simulink model "turbo_controller"  (R2025a)
settings: Solver=FixedStepAuto  StartTime=0.0  StopTime=inf  FixedStep=0.001  RelTol=1e-3
PostLoadFcn:
  | % 自动定位同目录CubeMX文件；不需要外部初始化脚本。
  | codertarget.data.setParameterValue('turbo_controller','STM32CubeMX.ProjectFile',fullfile(fileparts(get_param('turbo_controller','FileName')),'turbo_f407.ioc'));
InitFcn:
  | % 中文说明：按原控制器字段与类型创建三组接口总线；控制参数已内嵌。
  | tc_names=["EValve_Cycle" "EValve_Open" "Eblast_Cycle" "Eblast_Open" "Motor_Cycle" "Motor_Open" "EValve_Enable" "Eblast_Enable" "Motor_Enable" "SWO_Firework" "SWO_BleedAir" "EngineState" "Flag_ECUReset_Clear" "Flag_ECUReset_Save" "Flag_Reset_Enable" "Accelerator" "Nc_dem" "Nc"]; tc_types=["uint16" "uint16" "uint16" "uint16" "uint16" "uint16" "uint8" "uint8" "uint8" "uint8" "uint8" "uint8" "uint8" "uint8" "uint8" "single" "single" "single"];
  | for tc_k=1:numel(tc_names)
  |  tc_e(tc_k)=Simulink.BusElement; tc_e(tc_k).Name=char(tc_names(tc_k)); tc_e(tc_k).DataType=char(tc_types(tc_k));
  | end
  | EngineControl_Out=Simulink.Bus; EngineControl_Out.DataScope='Exported'; EngineControl_Out.Elements=tc_e;
  | clear tc_e tc_names tc_types tc_k
  | tc_names=["savedata1" "savedata2" "savedata3" "savedata4" "savedata5" "savedata6" "savedata7" "savedata8" "savedata9" "savedata10" "savedata11" "savedata12" "savedata13" "savedata14" "savedata15" "savedata16" "savedata17" "savedata18" "savedata19" "savedata20" "savedata21" "savedata22" "savedata23" "savedata24" "savedata25"]; tc_types=["single" "single" "single" "single" "single" "single" "single" "single" "single" "single" "single" "single" "single" "single" "single" "single" "single" "single" "single" "single" "single" "single" "single" "single" "single"];
  | for tc_k=1:numel(tc_names)
  |  tc_e(tc_k)=Simulink.BusElement; tc_e(tc_k).Name=char(tc_names(tc_k)); tc_e(tc_k).DataType=char(tc_types(tc_k));
  | end
  | SaveData_Out=Simulink.Bus; SaveData_Out.DataScope='Exported'; SaveData_Out.Elements=tc_e;
  | clear tc_e tc_names tc_types tc_k
  | tc_names=["senddata1" "senddata2" "senddata3" "senddata4" "senddata5" "senddata6" "senddata7" "senddata8" "senddata9" "senddata10" "senddata11" "senddata12" "senddata13" "senddata14" "senddata15" "senddata16" "senddata17" "senddata18" "senddata19" "senddata20" "senddata21" "senddata22" "senddata23" "senddata24" "senddata25" "senddata26" "senddata27" "senddata28" "senddata29"]; tc_types=["uint8" "uint8" "uint8" "uint8" "uint8" "uint8" "uint8" "uint8" "uint8" "uint8" "uint8" "uint8" "uint8" "uint8" "uint8" "uint8" "uint8" "uint8" "uint8" "uint8" "uint8" "uint8" "uint8" "uint8" "uint8" "uint8" "uint8" "uint8" "uint8"];
  | for tc_k=1:numel(tc_names)
  |  tc_e(tc_k)=Simulink.BusElement; tc_e(tc_k).Name=char(tc_names(tc_k)); tc_e(tc_k).DataType=char(tc_types(tc_k));
  | end
  | SendData_Out=Simulink.Bus; SendData_Out.DataScope='Exported'; SendData_Out.Elements=tc_e;
  | clear tc_e tc_names tc_types tc_k
  | 
  | % 以下为接口中文说明；只设置描述，不改变数值或数据类型。
  | EngineControl_Out.Description='执行控制输出（阀、电机、点火、状态及复位请求）';
  | tc_cn=["EValve_Cycle（主油阀周期计数（每计数2毫秒））" "EValve_Open（主油阀开通计数（每计数2毫秒））" "Eblast_Cycle（副油阀周期计数（每计数2毫秒））" "Eblast_Open（副油阀开通计数（每计数2毫秒））" "Motor_Cycle（起动电机周期计数）" "Motor_Open（起动电机开通计数）" "EValve_Enable（主油阀驱动使能）" "Eblast_Enable（副油阀驱动使能）" "Motor_Enable（起动电机使能）" "SWO_Firework（点火器使能（1开））" "SWO_BleedAir（引气阀使能（1开））" "EngineState（发动机状态）" "Flag_ECUReset_Clear（清除复位恢复状态请求）" "Flag_ECUReset_Save（保存复位恢复数据请求）" "Flag_Reset_Enable（处理器软件复位请求）" "Accelerator（油门／油泵给定控制量）" "Nc_dem（控制目标转速）" "Nc（发动机反馈转速（转每分））"];
  | tc_elements=EngineControl_Out.Elements;
  | for tc_k=1:numel(tc_cn)
  |  tc_elements(tc_k).Description=char(tc_cn(tc_k));
  | end
  | EngineControl_Out.Elements=tc_elements;
  | clear tc_cn tc_elements tc_k
  | SaveData_Out.Description='25项运行记录；字段含义按当前模型数据来源解释';
  | tc_cn=["savedata1（指令回显记录）" "savedata2（入口总温记录（℃））" "savedata3（电源电压记录）" "savedata4（排气温度记录（℃））" "savedata5（标定燃油压力记录）" "savedata6（副油阀占空比记录（％））" "savedata7（主油阀占空比记录（％））" "savedata8（温度修正转速记录）" "savedata9（开关输出及反馈位域）" "savedata10（物理转速记录）" "savedata11（油泵目标给定原始值）" "savedata12（起动电机占空比记录（％））" "savedata13（发动机状态码记录）" "savedata14（故障告警位域记录）" "savedata15（模型记录帧序号）" "savedata16（处理器温度记录（℃））" "savedata17（装订转速记录（沿用旧电源字段名））" "savedata18（导航高度记录）" "savedata19（飞行空速记录）" "savedata20（主阀旧记录位（恒零保留））" "savedata21（第21项保留记录（恒零））" "savedata22（保留记录项22）" "savedata23（保留记录项23）" "savedata24（保留记录项24）" "savedata25（保留记录项25）"];
  | tc_elements=SaveData_Out.Elements;
  | for tc_k=1:numel(tc_cn)
  |  tc_elements(tc_k).Description=char(tc_cn(tc_k));
  | end
  | SaveData_Out.Elements=tc_elements;
  | clear tc_cn tc_elements tc_k
  | SendData_Out.Description='29字段回传及外设命令接口；板端上位机帧只取第3至27字段';
  | tc_cn=["senddata1（回传发送允许标志（不直接上线路））" "senddata2（回传载荷长度25字节）" "senddata3（回传指令回显字节）" "senddata4（总温编码字节（℃＋80））" "senddata5（电源电压编码字节）" "senddata6（排温编码高字节）" "senddata7（排温编码低字节）" "senddata8（燃油压力编码高字节）" "senddata9（燃油压力编码低字节）" "senddata10（副油阀占空比字节（％））" "senddata11（主油阀占空比字节（％））" "senddata12（修正转速编码高字节）" "senddata13（修正转速编码低字节）" "senddata14（驱动及反馈状态位域）" "senddata15（物理转速编码高字节）" "senddata16（物理转速编码低字节）" "senddata17（油泵目标给定高字节（串口二使用））" "senddata18（油泵目标给定低字节（串口二使用））" "senddata19（起动电机占空比命令（串口一使用））" "senddata20（发动机状态码字节）" "senddata21（故障告警位域字节）" "senddata22（帧序号占位（板端另行填写））" "senddata23（处理器温度编码（℃＋50））" "senddata24（控制目标转速编码高字节）" "senddata25（控制目标转速编码低字节）" "senddata26（占位字节（板端改填实测泵速高字节））" "senddata27（占位字节（板端改填实测泵速低字节））" "senddata28（装订转速高字节（本板未发送））" "senddata29（装订转速低字节（本板未发送））"];
  | tc_elements=SendData_Out.Elements;
  | for tc_k=1:numel(tc_cn)
  |  tc_elements(tc_k).Description=char(tc_cn(tc_k));
  | end
  | SendData_Out.Elements=tc_elements;
  | clear tc_cn tc_elements tc_k
  | 
  | 
  | % FRAM模块化事务：接口类型和上电初始状态，随模型保存，无外部初始化文件。
  | clear FM_elements
  | FM_elements(1)=Simulink.BusElement;FM_elements(1).Name='phase';FM_elements(1).DataType='uint8';FM_elements(1).Dimensions=[1 1];FM_elements(1).Description='phase（当前事务阶段）';
  | FM_elements(2)=Simulink.BusElement;FM_elements(2).Name='a';FM_elements(2).DataType='uint8';FM_elements(2).Dimensions=[64 1];FM_elements(2).Description='a（启动时缓存的首区64字节）';
  | FM_elements(3)=Simulink.BusElement;FM_elements(3).Name='active';FM_elements(3).DataType='uint16';FM_elements(3).Dimensions=[1 1];FM_elements(3).Description='active（当前有效记录区地址）';
  | FM_elements(4)=Simulink.BusElement;FM_elements(4).Name='generation';FM_elements(4).DataType='uint32';FM_elements(4).Dimensions=[1 1];FM_elements(4).Description='generation（当前有效记录代号）';
  | FM_elements(5)=Simulink.BusElement;FM_elements(5).Name='record';FM_elements(5).DataType='uint8';FM_elements(5).Dimensions=[64 1];FM_elements(5).Description='record（本次冻结的待写记录）';
  | FM_elements(6)=Simulink.BusElement;FM_elements(6).Name='addr';FM_elements(6).DataType='uint16';FM_elements(6).Dimensions=[1 1];FM_elements(6).Description='addr（本次备用写入地址）';
  | FM_elements(7)=Simulink.BusElement;FM_elements(7).Name='lastSave';FM_elements(7).DataType='single';FM_elements(7).Dimensions=[1 1];FM_elements(7).Description='lastSave（上次开始保存的秒数）';
  | FM_elements(8)=Simulink.BusElement;FM_elements(8).Name='lastState';FM_elements(8).DataType='uint8';FM_elements(8).Dimensions=[1 1];FM_elements(8).Description='lastState（上次保存时的发动机状态）';
  | FM_elements(9)=Simulink.BusElement;FM_elements(9).Name='boot';FM_elements(9).DataType='boolean';FM_elements(9).Dimensions=[1 1];FM_elements(9).Description='boot（启动记录是否允许恢复）';
  | FM_elements(10)=Simulink.BusElement;FM_elements(10).Name='consumed';FM_elements(10).DataType='boolean';FM_elements(10).Dimensions=[1 1];FM_elements(10).Description='consumed（本次启动恢复通知是否已发送）';
  | FM_elements(11)=Simulink.BusElement;FM_elements(11).Name='payload';FM_elements(11).DataType='uint8';FM_elements(11).Dimensions=[20 1];FM_elements(11).Description='payload（当前20字节恢复内容）';
  | ... (+35 lines)
model workspace (MAT data in the model file):
  CRC16_Table_Reference = [0 4129 8258 12387 16516 20645 24774 28903 33032 37161 41290 45419 ... (256 elements, 256x1)]
  PE_Kaer = [0.15402 0.15402 0.12264 0.10076 0.09481 0.07601 0.07111 0.0569 0.05198 0.04926 0.05308 0.04325 ... (13 elements, 1x13)]
  PE_Nr = [21.2982 61.4260372 67.7475458 72.7394382 76.845934 80.6988798 83.8449282 86.6491912 88.9382406 89.178606 91.1938214 93.4068058 ... (13 elements, 1x13)]
  PE_Pump_Translate = 33.5999984741
  PE_RotaSpeed_Translate = 860
  PE_Taer = [0.4939154 0.4939154 0.40780982 0.34066978 0.31622756 0.30405716 0.34300244 0.26785022 0.37393554 0.23914836 0.44563948 0.31044662 ... (13 elements, 1x13)]
  PF_ACCFULLRANGE = 3360
  PF_Flag_ECUReset = 0
  PF_Flag_rx_suc = 1
  PF_Gear_Info = [40000; 45000; 50000; 55000; 57000; 59000; 60000; 61000; 61000; 61000; 61000; 61000]
  PF_K_TiaoJie = 1
  PF_Kpu = 10
  PF_MySet_Rxdata = [0 0 0 0 0 0 0 0 0 0 0 0 ... (50 elements, 50x1)]
  PF_MyUsart1_Rxdata = [0 0 0 0 0 0 0 0 0 0 0 0 ... (50 elements, 50x1)]
  PF_MyUsart2_Rxdata = [0 0 0 0 0 0 0 0 0 0 0 0 ... (50 elements, 50x1)]
  PF_Reset_Information = [0 0 0 0 0 0 0 0 0 0 0 0 ... (20 elements, 20x1)]
  PF_Sensor_X1_T4 = [0 4095]
  PF_Sensor_X2_T4 = [0 1.66666698456]
  PF_Sensor_X3_T4 = [0 504 999 1497 2010 2529 3051 3568 4076 4571 4959]
  PF_Sensor_X_P2 = [0.5 3]
  PF_Sensor_X_Poil = [0.5 3]
  PF_Sensor_X_T1t = [-50 300]
  PF_Sensor_X_Vpower = [0 3]
  PF_Sensor_X_Vpump = [0 3]
  PF_Sensor_Y1_T4 = [0 3]
  PF_Sensor_Y2_T4 = [0 5000]
  PF_Sensor_Y3_T4 = [0 100 200 300 400 500 600 700 800 900 980]
  PF_Sensor_Y_P2 = [0 1000]
  PF_Sensor_Y_Poil = [0 1000]
  PF_Sensor_Y_T1t = [-50 300]
  PF_Sensor_Y_Vpower = [0 33]
  PF_Sensor_Y_Vpump = [0 33]
  PG_CtrlMode_CloseLoop : mpt.Parameter (value not decoded)
  PG_CtrlMode_ManualAcc : mpt.Parameter (value not decoded)
  PG_CtrlMode_Origin : mpt.Parameter (value not decoded)
  PG_CtrlMode_Start : mpt.Parameter (value not decoded)
  PG_CtrlMode_Stop : mpt.Parameter (value not decoded)
  PG_ES_Clp : mpt.Parameter (value not decoded)
  PG_ES_EngStart : mpt.Parameter (value not decoded)
  PG_ES_Manual : mpt.Parameter (value not decoded)
  PG_ES_Origin : mpt.Parameter (value not decoded)
  PG_ES_Stop : mpt.Parameter (value not decoded)
  PG_Instr_BleedAirSet : mpt.Parameter (value not decoded)
  PG_Instr_CloseLoop : mpt.Parameter (value not decoded)
  PG_Instr_ECUReSet : mpt.Parameter (value not decoded)
  PG_Instr_EValveSet : mpt.Parameter (value not decoded)
  PG_Instr_EblastSet : mpt.Parameter (value not decoded)
  PG_Instr_Erase : mpt.Parameter (value not decoded)
  PG_Instr_FireWorkSet : mpt.Parameter (value not decoded)
  PG_Instr_ManualPlus : mpt.Parameter (value not decoded)
  PG_Instr_ManualrReduce : mpt.Parameter (value not decoded)
  PG_Instr_MotorSet : mpt.Parameter (value not decoded)
  PG_Instr_OilSet : mpt.Parameter (value not decoded)
  PG_Instr_SelfCheck : mpt.Parameter (value not decoded)
  PG_Instr_Start : mpt.Parameter (value not decoded)
  PG_Instr_Stop : mpt.Parameter (value not decoded)
  PG_Instr_StopZero : Simulink.Parameter (value not decoded)
  PG_Location_Air : Simulink.Parameter (value not decoded)
  PG_Location_Gnd : Simulink.Parameter (value not decoded)
  PG_ServoCtrlMode_CloseLoop : Simulink.Parameter (value not decoded)
  PG_ServoCtrlMode_CloseLoopMax : Simulink.Parameter (value not decoded)
  PG_ServoCtrlMode_CloseLoopMin : Simulink.Parameter (value not decoded)
  PG_ServoCtrlMode_ManualAcc : Simulink.Parameter (value not decoded)
  PG_ServoCtrlMode_ManualAccMax : Simulink.Parameter (value not decoded)
  PG_ServoCtrlMode_ManualAccMin : Simulink.Parameter (value not decoded)
  PG_SpeedDot_Permit : Simulink.Parameter (value not decoded)
  PL_EngineModel_Actuator = [0 10 100]
  PL_EngineModel_EngineStar_Press_P2 = [1013 1098.4 1099.144828 1099.931034 1103.613793 1162.662069 1143.793103 1131.006897 1123.186207 1117.6 1114 1111.806897 ... (127 elements, 1x127)]
  PL_EngineModel_EngineStar_RotaSpeed = [200 2000 9584 9660 10220 10240 10260 10288 10308 10368 10380 10408 ... (127 elements, 1x127)]
  PL_EngineModel_EngineStar_Temp_Exhaust = [128 129 129.1 130 131 131.1 132 133 134 134.1 135 135.1 ... (127 elements, 1x127)]
  PL_EngineModel_EngineStar_Time = [0.05 0.1 0.15 0.2 0.25 0.3 0.35 0.4 0.45 0.5 0.55 0.6 ... (127 elements, 1x127)]
  PL_EngineModel_IdleAbove_Nr = [0 21.2982 61.4260372 67.7475458 72.7394382 76.845934 80.6988798 83.8449282 86.6491912 88.9382406 89.178606 91.1938214 ... (14 elements, 1x14)]
  PL_EngineModel_IdleAbove_P2r = [0.986923266716 1.57907722675 1.81593881076 1.99358499877 2.23044658278 2.43770046879 2.65482358747 2.84233900814 3.03972366149 3.18776215149 3.25684678016 3.3950160375 ... (14 elements, 1x14)]
  PL_EngineModel_IdleAbove_Tempr = [0.0536001429337 1.07200285867 1.63301768805 1.63659103091 1.66875111667 1.72592460247 1.77595140254 1.86171163123 1.95461854565 2.03323208862 2.03323208862 2.13685903162 ... (14 elements, 1x14)]
  PL_EngineModel_IdleAbove_Ter = [0.42434128 0.42434128 0.42434128 0.30669408 0.23570008 0.22150128 0.1997974 0.23803274 0.16115638 0.24279948 0.13600422 0.31308354 ... (14 elements, 1x14)]
  PL_EngineModel_IdleAbove_Wfr = [0 10.142 23.8337 27.8905 31.9473 36.0041 40.0609 44.1177 48.1745 52.2313 52.7384 56.7952 ... (14 elements, 1x14)]
  PL_EngineModel_Press_P2 = [400 400 400 400 400 400 400 400 400 400]
  PL_EngineModel_Rotaspeed = [0 20000 96400]
  PL_EngineModel_Temp_Exhaust = [500 500 500 500 500 500 500 500 500 500]
  PL_Kaer = [0.1 0.1 0.1 0.1 0.1 0.1]
  PL_Nr = [50 60 70 80 90 100]
  PL_Taer = [0.1 0.1 0.1 0.1 0.1 0.1]
  Sig : Simulink.Signal (value not decoded)
  Ts_ms : Simulink.Parameter (value not decoded)
  false : Simulink.Parameter (value not decoded)
  true : Simulink.Parameter (value not decoded)
symbols that are objects in the model workspace (value not decoded): PG_CtrlMode_CloseLoop, PG_CtrlMode_ManualAcc, PG_CtrlMode_Origin, PG_CtrlMode_Start, PG_CtrlMode_Stop, PG_ES_Clp, PG_ES_EngStart, PG_ES_Manual, PG_ES_Origin, PG_ES_Stop, PG_Instr_BleedAirSet, PG_Instr_CloseLoop, PG_Instr_EblastSet, PG_Instr_ECUReSet, PG_Instr_Erase, PG_Instr_EValveSet, PG_Instr_FireWorkSet, PG_Instr_ManualPlus, PG_Instr_ManualrReduce, PG_Instr_MotorSet, PG_Instr_OilSet, PG_Instr_SelfCheck, PG_Instr_Start, PG_Instr_Stop, PG_Instr_StopZero, PG_ServoCtrlMode_CloseLoop, PG_ServoCtrlMode_CloseLoopMax, PG_ServoCtrlMode_CloseLoopMin, PG_ServoCtrlMode_ManualAcc, PG_ServoCtrlMode_ManualAccMax, PG_ServoCtrlMode_ManualAccMin, Ts_ms
libraries: simulink x97, stm32blockslib x10, stm32f4xxblockslib x8
(part 3 of 26)

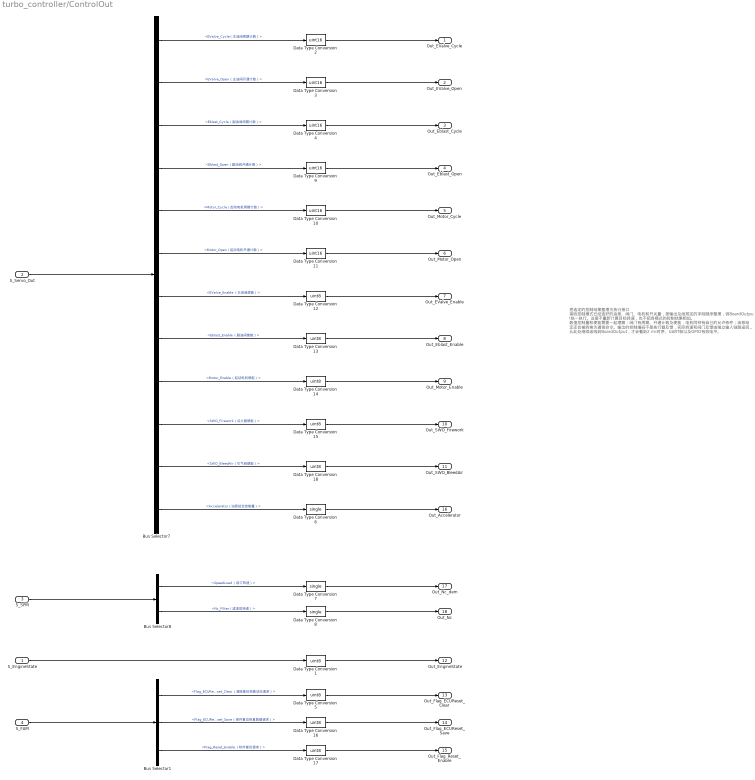
== system turbo_controller/ControlOut ==
  note: 把选定的控制结果整理为执行接口
      |
      | 接收控制模式已经选好的油泵、阀门、电机和开关量，按输出总线规定的字段顺序整理，供BoardOutpu
      | t统一执行。这里不重新计算目标转速，也不把各模式的控制结果相加。
      |
      | 数值控制量和使能需要一起理解：阀门有周期、开通计数及使能，电机同样有自己的允许条件；油泵给
      | 定还会被转换为通信命令。输出的控制编码不是执行器反馈，实际转速和阀门反馈由独立输入链路返回
      | 。
      |
      | 从此处继续追线到BoardOutput，才会看到2 ms时序、UART帧以及GPIO有效电平。
  S_EngineState : Inport
      settings: AttributesFormatString=S_EngineState（发动机状态）
  S_Servo_Out : Inport  Port=2
      settings: AttributesFormatString=S_Servo_Out（伺服输出）
  S_SPM : Inport  Port=3
      settings: AttributesFormatString=S_SPM（通信及传感器信息总线）
  S_FAM : Inport  Port=4
      settings: AttributesFormatString=S_FAM（故障标志总线）
  Bus Selector1 : BusSelector  OutputSignals=Flag_ECUReset_Clear（清除复位恢复状态请求）,Flag_ECUReset_Save（保存复位恢复数据请求）,Flag_Reset_Enable（软件复位请求）
      settings: AttributesFormatString=Bus Selector1（总线选择器1）
  Bus Selector7 : BusSelector  OutputSignals=EValve_Cycle（主油阀周期计数）,EValve_Open（主油阀开通计数）,Eblast_Cycle（副油阀周期计数）,Eblast_Open（副油阀开通计数）,Motor_Cycle（起动电机周期计数）,Motor_Open（起动电机开通计数）,EValve_Enable（主油阀使能）,Eblast_Enable（副油阀使能）,Motor_Enable（起动电机使能）,SWO_Firework（点火器使能）,SWO_BleedAir（引气阀使能）,Accelerator（油泵给定控制量）
      settings: AttributesFormatString=Bus Selector7（总线选择器7）
  Bus Selector8 : BusSelector  OutputSignals=COMM（通信信息总线）.SpeedLoad（装订转速）,Sensor（传感器信息总线）.Nc_Filter（滤波后转速）
      settings: AttributesFormatString=Bus Selector8（总线选择器8）
  Data Type Conversion{1,5,12..18} (9 alike) : DataTypeConversion  OutDataTypeStr=uint8  SaturateOnIntegerOverflow=off  RndMeth=Floor
      Data Type Conversion1 settings: AttributesFormatString=Data Type Conversion1（数据类型转换1）
      Data Type Conversion12 settings: AttributesFormatString=Data Type Conversion12（数据类型转换12）
      Data Type Conversion13 settings: AttributesFormatString=Data Type Conversion13（数据类型转换13）
      Data Type Conversion14 settings: AttributesFormatString=Data Type Conversion14（数据类型转换14）
      Data Type Conversion15 settings: AttributesFormatString=Data Type Conversion15（数据类型转换15）
      Data Type Conversion16 settings: AttributesFormatString=Data Type Conversion16（数据类型转换16）
      Data Type Conversion17 settings: AttributesFormatString=Data Type Conversion17（数据类型转换17）
      Data Type Conversion18 settings: AttributesFormatString=Data Type Conversion18（数据类型转换18）
      Data Type Conversion5 settings: AttributesFormatString=Data Type Conversion5（数据类型转换5）
  Data Type Conversion{2..4,9..11} (6 alike) : DataTypeConversion  OutDataTypeStr=uint16  SaturateOnIntegerOverflow=off  RndMeth=Floor
      Data Type Conversion10 settings: AttributesFormatString=Data Type Conversion10（数据类型转换10）
      Data Type Conversion11 settings: AttributesFormatString=Data Type Conversion11（数据类型转换11）
      Data Type Conversion2 settings: AttributesFormatString=Data Type Conversion2（数据类型转换2）
      Data Type Conversion3 settings: AttributesFormatString=Data Type Conversion3（数据类型转换3）
      Data Type Conversion4 settings: AttributesFormatString=Data Type Conversion4（数据类型转换4）
      Data Type Conversion9 settings: AttributesFormatString=Data Type Conversion9（数据类型转换9）
  Data Type Conversion6 : DataTypeConversion  OutDataTypeStr=single  SaturateOnIntegerOverflow=off  RndMeth=Floor
      settings: AttributesFormatString=Data Type Conversion6（数据类型转换6）
  Data Type Conversion7 : DataTypeConversion  OutDataTypeStr=single  SaturateOnIntegerOverflow=off  RndMeth=Floor
      settings: AttributesFormatString=Data Type Conversion7（数据类型转换7）
  Data Type Conversion8 : DataTypeConversion  OutDataTypeStr=single  SaturateOnIntegerOverflow=off  RndMeth=Floor
      settings: AttributesFormatString=Data Type Conversion8（数据类型转换8）
  Out_EValve_Cycle : Outport
      settings: AttributesFormatString=Out_EValve_Cycle（主油阀周期计数（每计数2毫秒））
  Out_EValve_Open : Outport  Port=2
      settings: AttributesFormatString=Out_EValve_Open（主油阀开通计数（每计数2毫秒））
  Out_Eblast_Cycle : Outport  Port=3
      settings: AttributesFormatString=Out_Eblast_Cycle（副油阀周期计数（每计数2毫秒））
  Out_Eblast_Open : Outport  Port=4
      settings: AttributesFormatString=Out_Eblast_Open（副油阀开通计数（每计数2毫秒））
  Out_Motor_Cycle : Outport  Port=5
      settings: AttributesFormatString=Out_Motor_Cycle（起动电机周期计数）
  Out_Motor_Open : Outport  Port=6
      settings: AttributesFormatString=Out_Motor_Open（起动电机开通计数）
  Out_EValve_Enable : Outport  Port=7
      settings: AttributesFormatString=Out_EValve_Enable（主油阀驱动使能）
  Out_Eblast_Enable : Outport  Port=8
      settings: AttributesFormatString=Out_Eblast_Enable（副油阀驱动使能）
  Out_Motor_Enable : Outport  Port=9
      settings: AttributesFormatString=Out_Motor_Enable（起动电机使能）
  Out_SWO_Firework : Outport  Port=10
      settings: AttributesFormatString=Out_SWO_Firework（点火器使能（1开））
  Out_SWO_BleedAir : Outport  Port=11
      settings: AttributesFormatString=Out_SWO_BleedAir（引气阀使能（1开））
  Out_EngineState : Outport  Port=12
      settings: AttributesFormatString=Out_EngineState（发动机状态）
  Out_Flag_ECUReset_Clear : Outport  Port=13
      settings: AttributesFormatString=Out_Flag_ECUReset_Clear（清除复位恢复状态请求）
  Out_Flag_ECUReset_Save : Outport  Port=14
      settings: AttributesFormatString=Out_Flag_ECUReset_Save（保存复位恢复数据请求）
  Out_Flag_Reset_Enable : Outport  Port=15
      settings: AttributesFormatString=Out_Flag_Reset_Enable（处理器软件复位请求）
  Out_Accelerator : Outport  Port=16
      settings: AttributesFormatString=Out_Accelerator（油门／油泵给定控制量）
  Out_Nc_dem : Outport  Port=17
      settings: AttributesFormatString=Out_Nc_dem（控制目标转速）
  Out_Nc : Outport  Port=18
      settings: AttributesFormatString=Out_Nc（发动机反馈转速（转每分））
  wires:
  S_Servo_Out/1 -> Bus Selector7/1
  S_EngineState/1 -> Data Type Conversion1/1
  Bus Selector8/1 -> Data Type Conversion7/1  "<SpeedLoad（装订转速）>"
  Bus Selector1/1 -> Data Type Conversion5/1  "<Flag_ECUReset_Clear（清除复位恢复状态请求）>"
  Data Type Conversion1/1 -> Out_EngineState/1
  Data Type Conversion2/1 -> Out_EValve_Cycle/1
  Data Type Conversion5/1 -> Out_Flag_ECUReset_Clear/1
  Data Type Conversion6/1 -> Out_Accelerator/1
  Bus Selector8/2 -> Data Type Conversion8/1  "<Nc_Filter（滤波后转速）>"
  Data Type Conversion7/1 -> Out_Nc_dem/1
  Data Type Conversion8/1 -> Out_Nc/1
  S_SPM/1 -> Bus Selector8/1
  Bus Selector7/1 -> Data Type Conversion2/1  "<EValve_Cycle（主油阀周期计数）>"
  Bus Selector7/12 -> Data Type Conversion6/1  "<Accelerator（油泵给定控制量）>"
  Bus Selector7/2 -> Data Type Conversion3/1  "<EValve_Open（主油阀开通计数）>"
  Bus Selector7/3 -> Data Type Conversion4/1  "<Eblast_Cycle（副油阀周期计数）>"
  Bus Selector7/4 -> Data Type Conversion9/1  "<Eblast_Open（副油阀开通计数）>"
  Bus Selector7/5 -> Data Type Conversion10/1  "<Motor_Cycle（起动电机周期计数）>"
  Bus Selector7/7 -> Data Type Conversion12/1  "<EValve_Enable（主油阀使能）>"
  Bus Selector7/8 -> Data Type Conversion13/1  "<Eblast_Enable（副油阀使能）>"
  Bus Selector7/9 -> Data Type Conversion14/1  "<Motor_Enable（起动电机使能）>"
  Bus Selector7/10 -> Data Type Conversion15/1  "<SWO_Firework（点火器使能）>"
  Data Type Conversion3/1 -> Out_EValve_Open/1
  Data Type Conversion4/1 -> Out_Eblast_Cycle/1
  Data Type Conversion9/1 -> Out_Eblast_Open/1
  Data Type Conversion10/1 -> Out_Motor_Cycle/1
  Data Type Conversion11/1 -> Out_Motor_Open/1
  Data Type Conversion12/1 -> Out_EValve_Enable/1
  Data Type Conversion13/1 -> Out_Eblast_Enable/1
  Data Type Conversion14/1 -> Out_Motor_Enable/1
  Data Type Conversion15/1 -> Out_SWO_Firework/1
  S_FAM/1 -> Bus Selector1/1
  Data Type Conversion16/1 -> Out_Flag_ECUReset_Save/1
  Bus Selector1/2 -> Data Type Conversion16/1  "<Flag_ECUReset_Save（保存复位恢复数据请求）>"
  Bus Selector1/3 -> Data Type Conversion17/1  "<Flag_Reset_Enable（软件复位请求）>"
  Data Type Conversion17/1 -> Out_Flag_Reset_Enable/1
  Data Type Conversion18/1 -> Out_SWO_BleedAir/1
  Bus Selector7/11 -> Data Type Conversion18/1  "<SWO_BleedAir（引气阀使能）>"
  Bus Selector7/6 -> Data Type Conversion11/1  "<Motor_Open（起动电机开通计数）>"

== system turbo_controller/ESM ==
  note: 管理发动机运行模式，而不是直接控制驱动电平
      |
      | Flags先根据命令、当前转速、起动阶段结果、停车完成标志及恢复条件，计算允许发生哪些模式转换
      | 。StateTranslation再按当前所在模式和这些允许条件切换状态。
      |
      | 对外只有五种运行模式：Origin=0、Start=1、Clp=2、Manual=3、Stop=4。普通起动内部的A～F及异常
      | 阶段码不属于这五个模式编号。
      |
      | 输出EngineState供CLM选择相应控制分支，供通信与记录解释运行状态。本层不生成泵字节或GPIO脉冲
      | ；转换进入Start仅表示开始执行起动分支，不代表已达到闭环转速。
  S_CLM_Parameter : Inport
      settings: AttributesFormatString=S_CLM_Parameter（控制规律管理模块参数）
  S_SPM : Inport  Port=2
      settings: AttributesFormatString=S_SPM（通信及传感器信息总线）
  Bus Selector1 : BusSelector  OutputSignals=Sensor（传感器信息总线）.Nc_Filter（滤波后转速）,COMM（通信信息总线）.Instr（控制指令）,COMM（通信信息总线）.Flag_ECUReset_Use（复位恢复数据使用标志）
      settings: AttributesFormatString=Bus Selector1（总线选择器1）
  Flags : Subsystem  Description=|  RequirementInfo={} %GIDa_327e6870_9dda_480b_a4d4_89db54ff38ee  RTWFileName=MCM_FPM
      | 把分散的进入条件整理为11个模式转换标志
      | 
      | 分别检查初始到起动、初始到手动、进入闭环、各模式停车、停车回初始等条件，再将11个布尔结果打成Flags总线交状态机使用。
      | 
      | 例如普通起动要求Start命令且转速不超过13000；停车回初始要求停车完成且转速不超过20000。部分控制分支结果先经过一拍延迟再反馈，防止同一拍组合判断互相循环。
      | 
      | 这里的每一项是“是否允许这条转换”，不是发动机模式本身，也不是报警编号。真正的当前模式由StateTranslation保存。
      settings: AttributesFormatString=Flags（标志集合）  RTWSystemCode=Nonreusable function  RTWFcnNameOpts=Use subsystem name  RTWFileNameOpts=User specified
  StateTransition : Subsystem  Description=|  RequirementInfo={} %GIDa_4be7af36_387d_4f9f_aca0_47de2d8959f7  TreatAsAtomicUnit=on  RTWFileName=MCM_FPM
      | 管理发动机运行模式，而不是直接控制驱动电平
      | 
      | Flags先根据命令、当前转速、起动阶段结果、停车完成标志及恢复条件，计算允许发生哪些模式转换。StateTranslation再按当前所在模式和这些允许条件切换状态。
      | 
      | 对外只有五种运行模式：Origin=0、Start=1、Clp=2、Manual=3、Stop=4。普通起动内部的A～F及异常阶段码不属于这五个模式编号。
      | 
      | 输出EngineState供CLM选择相应控制分支，供通信与记录解释运行状态。本层不生成泵字节或GPIO脉冲；转换进入Start仅表示开始执行起动分支，不代表已达到闭环转速。
      settings: AttributesFormatString=StateTransition（状态转换管理）  RTWFcnNameOpts=Use subsystem name  RTWFileNameOpts=User specified
  S_EngineState : Outport
      settings: AttributesFormatString=S_EngineState（发动机状态）
  wires:
  S_SPM/1 -> Bus Selector1/1
  Flags/1(S_Flags) -> StateTransition/1(S_Flags)
  StateTransition/1(S_EngineState) -> S_EngineState/1
  Bus Selector1/1 -> Flags/1(S_Nc)  "<Nc_Filter（滤波后转速）>"
  Bus Selector1/2 -> Flags/2(S_Instr)  "<Instr（控制指令）>"
  Bus Selector1/3 -> Flags/3(S_Flag_ECUReset)  "<Flag_ECUReset_Use（复位恢复数据使用标志）>"
  S_CLM_Parameter/1 -> Flags/4(S_CLM_Parameter)

== system turbo_controller/FPM ==
  note: 【本页库子系统中文说明】停车状态
      | 一、它做什么？
      | 这是“过不过这条线”的判断器。将输入与阈值 PG_ES_Stop 作 == 比较，关系成立输
      | 出真（1），否则输出假（0）。例如>=包含恰好等于，>则不包含。它只给出判断标志
      | ，不会自行限幅、报警、切换状态或操作阀门；后续逻辑决定如何使用。名称可能只是
      | 用途提示，实际判据以这里的关系和阈值为准。
      | 二、本实例当前参数
      | 比较关系：==
      | 比较阈值：PG_ES_Stop
      | 输出数据类型：uint8
      | 零交叉检测：开启
      | 三、怎样继续学习？
      | 这是标准库子系统实例。中文说明放在使用它的父级页面，并同步存入本块Descriptio
      | n（模块说明）；官方库链接保留。先看本实例的输入来自哪里、输出交给谁，再结合
      | 以上参数理解作用。
  note: 【本页库子系统中文说明】初始状态
      | 一、它做什么？
      | 这是“过不过这条线”的判断器。将输入与阈值 PG_ES_Origin 作 == 比较，关系成立
      | 输出真（1），否则输出假（0）。例如>=包含恰好等于，>则不包含。它只给出判断标
      | 志，不会自行限幅、报警、切换状态或操作阀门；后续逻辑决定如何使用。名称可能只
      | 是用途提示，实际判据以这里的关系和阈值为准。
      | 二、本实例当前参数
      | 比较关系：==
      | 比较阈值：PG_ES_Origin
      | 输出数据类型：uint8
      | 零交叉检测：开启
      | 三、怎样继续学习？
      | 这是标准库子系统实例。中文说明放在使用它的父级页面，并同步存入本块Descriptio
      | n（模块说明）；官方库链接保留。先看本实例的输入来自哪里、输出交给谁，再结合
      | 以上参数理解作用。
  note: 【本页库子系统中文说明】手动
      | 一、它做什么？
      | 这是“过不过这条线”的判断器。将输入与阈值 PG_ES_Manual 作 == 比较，关系成立
      | 输出真（1），否则输出假（0）。例如>=包含恰好等于，>则不包含。它只给出判断标
      | 志，不会自行限幅、报警、切换状态或操作阀门；后续逻辑决定如何使用。名称可能只
      | 是用途提示，实际判据以这里的关系和阈值为准。
      | 二、本实例当前参数
      | 比较关系：==
      | 比较阈值：PG_ES_Manual
      | 输出数据类型：uint8
      | 零交叉检测：开启
      | 三、怎样继续学习？
      | 这是标准库子系统实例。中文说明放在使用它的父级页面，并同步存入本块Descriptio
      | n（模块说明）；官方库链接保留。先看本实例的输入来自哪里、输出交给谁，再结合
      | 以上参数理解作用。
  note: 【本页库子系统中文说明】起动
      | 一、它做什么？
      | 这是“过不过这条线”的判断器。将输入与阈值 PG_ES_EngStart 作 == 比较，关系成
      | 立输出真（1），否则输出假（0）。例如>=包含恰好等于，>则不包含。它只给出判断
      | 标志，不会自行限幅、报警、切换状态或操作阀门；后续逻辑决定如何使用。名称可能
      | 只是用途提示，实际判据以这里的关系和阈值为准。
      | 二、本实例当前参数
      | 比较关系：==
      | 比较阈值：PG_ES_EngStart
      | 输出数据类型：uint8
      | 零交叉检测：开启
      | 三、怎样继续学习？
      | 这是标准库子系统实例。中文说明放在使用它的父级页面，并同步存入本块Descriptio
      | n（模块说明）；官方库链接保留。先看本实例的输入来自哪里、输出交给谁，再结合
      | 以上参数理解作用。
  note: 【本页库子系统中文说明】超转保护
      | 一、它做什么？
      | 这是“过不过这条线”的判断器。将输入与阈值 62000 作 > 比较，关系成立输出真（
      | 1），否则输出假（0）。例如>=包含恰好等于，>则不包含。它只给出判断标志，不会
      | 自行限幅、报警、切换状态或操作阀门；后续逻辑决定如何使用。名称可能只是用途提
      | 示，实际判据以这里的关系和阈值为准。
      | 二、本实例当前参数
      | 比较关系：>
      | 比较阈值：62000
      | 输出数据类型：uint8
      | 零交叉检测：开启
      | 三、怎样继续学习？
      | 这是标准库子系统实例。中文说明放在使用它的父级页面，并同步存入本块Descriptio
      | n（模块说明）；官方库链接保留。先看本实例的输入来自哪里、输出交给谁，再结合
      | 以上参数理解作用。
  note: 【本页库子系统中文说明】重置指令
      | 一、它做什么？
      | 这是“过不过这条线”的判断器。将输入与阈值 PG_Instr_ECUReSet 作 == 比较，关
      | 系成立输出真（1），否则输出假（0）。例如>=包含恰好等于，>则不包含。它只给出
      | 判断标志，不会自行限幅、报警、切换状态或操作阀门；后续逻辑决定如何使用。名称
      | 可能只是用途提示，实际判据以这里的关系和阈值为准。
      | 二、本实例当前参数
      | 比较关系：==
      | 比较阈值：PG_Instr_ECUReSet
      | 输出数据类型：uint8
      | 零交叉检测：开启
      | 三、怎样继续学习？
      | 这是标准库子系统实例。中文说明放在使用它的父级页面，并同步存入本块Descriptio
      | n（模块说明）；官方库链接保留。先看本实例的输入来自哪里、输出交给谁，再结合
      | 以上参数理解作用。
  note: 【本页库子系统中文说明】闭环
      | 一、它做什么？
      | 这是“过不过这条线”的判断器。将输入与阈值 PG_ES_Clp 作 == 比较，关系成立输
      | 出真（1），否则输出假（0）。例如>=包含恰好等于，>则不包含。它只给出判断标志
      | ，不会自行限幅、报警、切换状态或操作阀门；后续逻辑决定如何使用。名称可能只是
      | 用途提示，实际判据以这里的关系和阈值为准。
      | 二、本实例当前参数
      | 比较关系：==
      | 比较阈值：PG_ES_Clp
      | 输出数据类型：uint8
      | 零交叉检测：开启
      | 三、怎样继续学习？
      | 这是标准库子系统实例。中文说明放在使用它的父级页面，并同步存入本块Descriptio
      | n（模块说明）；官方库链接保留。先看本实例的输入来自哪里、输出交给谁，再结合
      | 以上参数理解作用。
  note: 将测速异常和复位请求整理成控制保护标志
      |
      | 从传感器和通信总线取得转速、故障状态、命令及运行模式。内部区分暂时的测速异常、持续故障锁存
      | ，以及恢复、清除和定期保存条件。
      |
      | 转速超过62000的比较参与手动超速保护；ECUReset命令经Up_Hold保持，结合模式形成复位相关请求。
      | 输出FAM总线供CLM选择保持原泵值、备份供油曲线或恢复期间给定，并送FRAM事务层保存。
      |
      | 本模块主要生成逻辑条件，不直接写FRAM或调用硬件复位。故障标志成立后的实际控制策略，在CLM/Fa
      | ult_Process和输出管理中实现。
  note: 停车状态
      | 停车状态：只判断一个条件
      |
      | 把输入与4比较，使用关系“==”。成立输出1，不成立输出0；输出是判断标志，不是把输入缩放成该
      | 常数。
      |
      | 这里比较的是发动机当前模式：初始0、普通起动1、闭环2、手动3、停车4。结果供父级选择对应控制/
      | 保护路径，不能用命令编号代替模式编号。
  note: 初始状态
      | 初始状态：只判断一个条件
      |
      | 把输入与0比较，使用关系“==”。成立输出1，不成立输出0；输出是判断标志，不是把输入缩放成该
      | 常数。
      |
      | 这里比较的是发动机当前模式：初始0、普通起动1、闭环2、手动3、停车4。结果供父级选择对应控制/
      | 保护路径，不能用命令编号代替模式编号。
  note: 手动
      | 手动：只判断一个条件
      |
      | 把输入与3比较，使用关系“==”。成立输出1，不成立输出0；输出是判断标志，不是把输入缩放成该
      | 常数。
      |
      | 这里比较的是发动机当前模式：初始0、普通起动1、闭环2、手动3、停车4。结果供父级选择对应控制/
      | 保护路径，不能用命令编号代替模式编号。
  note: 起动
      | 起动：只判断一个条件
      |
      | 把输入与1比较，使用关系“==”。成立输出1，不成立输出0；输出是判断标志，不是把输入缩放成该
      | 常数。
      |
      | 这里比较的是发动机当前模式：初始0、普通起动1、闭环2、手动3、停车4。结果供父级选择对应控制/
      | 保护路径，不能用命令编号代替模式编号。
  note: 超转保护
      | 超转保护：只判断一个条件
      |
      | 把输入与62000比较，使用关系“>”。成立输出1，不成立输出0；输出是判断标志，不是把输入缩放成
      | 该常数。
      |
      | 比较门限用于父级的分支条件，没有滤波、延时确认或锁存。例如输入恰好等于门限时，“>=、<=、==
      | ”成立，“>、<”不成立。是否需要持续确认或同时满足其他条件，由父级连线决定。
  note: 重置指令
      | 重置指令：只判断一个条件
      |
      | 把输入与9比较，使用关系“==”。成立输出1，不成立输出0；输出是判断标志，不是把输入缩放成该
      | 常数。
      |
      | 这里识别一种指令编码。判断成立只说明指令匹配；父级还会结合有效帧、当前模式或其他允许条件决
      | 定是否更新。实际驱动要继续经过控制与板级输出，不能把1理解为硬件执行回执。
  note: 闭环
      | 闭环：只判断一个条件
      |
      | 把输入与2比较，使用关系“==”。成立输出1，不成立输出0；输出是判断标志，不是把输入缩放成该
      | 常数。
      |
      | 这里比较的是发动机当前模式：初始0、普通起动1、闭环2、手动3、停车4。结果供父级选择对应控制/
      | 保护路径，不能用命令编号代替模式编号。
  S_SPM : Inport
      settings: AttributesFormatString=S_SPM（通信及传感器信息总线）
  S_EngineState : Inport  Port=2
      settings: AttributesFormatString=S_EngineState（发动机状态）
  Bus Creator1 : BusCreator  Inputs=8
      settings: AttributesFormatString=Bus Creator1（总线创建器1）
  Bus Selector1 : BusSelector  OutputSignals=Sensor（传感器信息总线）.Nc_Filter（滤波后转速）
      settings: AttributesFormatString=Bus Selector1（总线选择器1）
  Bus Selector2 : BusSelector  OutputSignals=COMM（通信信息总线）.Instr（控制指令）
      settings: AttributesFormatString=Bus Selector2（总线选择器2）
  Data Type Conversion1 : DataTypeConversion  OutDataTypeStr=uint8  SaturateOnIntegerOverflow=off  RndMeth=Floor
      settings: AttributesFormatString=Data Type Conversion1（数据类型转换1）
  Data Type Conversion2 : DataTypeConversion  OutDataTypeStr=uint8  SaturateOnIntegerOverflow=off  RndMeth=Floor
      settings: AttributesFormatString=Data Type Conversion2（数据类型转换2）
  Logical Operator1 : Logic  Operator=OR  AllPortsSameDT=off  OutDataTypeStr=boolean
      settings: AttributesFormatString=Logical Operator1（逻辑运算1）
  Logical Operator2 : Logic  Inputs=3  AllPortsSameDT=off  OutDataTypeStr=boolean
      settings: AttributesFormatString=Logical Operator2（逻辑运算2）
  Logical Operator3 : Logic  Operator=OR  Inputs=3  AllPortsSameDT=off  OutDataTypeStr=boolean
      settings: AttributesFormatString=Logical Operator3（逻辑运算3）
  Subsystem : Subsystem  Description=|
      | 区分短时测速异常、持续故障和恢复保存时机
      | 
      | 把转速幅值故障与突变故障组合，先形成当前异常，再经10 s定时锁存形成持续故障。暂时异常可让控制保持，持续异常则允许父级切换备份供油策略。
      | 
      | 恢复有效条件持续约2 s后产生恢复工作相关状态；处于闭环时，4 s计时器周期性给出保存事件。模式变化检测与触发/使能分支产生恢复信息清除请求。
      | 
      | 这些都是控制条件，不是FRAM写入已完成的确认。实际保存需要下游事务逐步执行，写失败也不能仅靠本模块得知。
      settings: AttributesFormatString=Subsystem（子系统）
  Up_Hold : Stateflow chart  Description=|  TreatAsAtomicUnit=on  RTWFcnName=Timmer  RTWFileName=EngineControl_Timmer
      | 把复位请求锁住，避免一拍命令丢失
      | 
      | 输入In一旦为真，就把Out置为真。图内没有输入变假就清Out的对应动作，因此它是请求锁存，而不是简单复制输入，也不是单拍脉冲。
      | 
      | 后续模式与事务逻辑可以在命令消失后继续看到请求。锁存状态在模型或图初始化时重置；此图不等待SPI完成，也不表示硬件复位已经执行。
      settings: AttributesFormatString=Up_Hold（上升或增加保持）  RTWSystemCode=Reusable function  RTWFcnNameOpts=Use subsystem name  RTWFileNameOpts=User specified
  停车状态 : simulink/Logic and Bit Operations/Compare To Constant  Description=|  relop===  const=PG_ES_Stop  OutDataTypeStr=uint8
      | 停车状态：只判断一个条件
      | 
      | 把输入与4比较，使用关系“==”。成立输出1，不成立输出0；输出是判断标志，不是把输入缩放成该常数。
      | 
      | 这里比较的是发动机当前模式：初始0、普通起动1、闭环2、手动3、停车4。结果供父级选择对应控制/保护路径，不能用命令编号代替模式编号。
  初始状态 : simulink/Logic and Bit Operations/Compare To Constant  Description=|  relop===  const=PG_ES_Origin  OutDataTypeStr=uint8
      | 初始状态：只判断一个条件
      | 
      | 把输入与0比较，使用关系“==”。成立输出1，不成立输出0；输出是判断标志，不是把输入缩放成该常数。
      | 
      | 这里比较的是发动机当前模式：初始0、普通起动1、闭环2、手动3、停车4。结果供父级选择对应控制/保护路径，不能用命令编号代替模式编号。
  手动 : simulink/Logic and Bit Operations/Compare To Constant  Description=|  relop===  const=PG_ES_Manual  OutDataTypeStr=uint8
      | 手动：只判断一个条件
      | 
      | 把输入与3比较，使用关系“==”。成立输出1，不成立输出0；输出是判断标志，不是把输入缩放成该常数。
      | 
      | 这里比较的是发动机当前模式：初始0、普通起动1、闭环2、手动3、停车4。结果供父级选择对应控制/保护路径，不能用命令编号代替模式编号。
  起动 : simulink/Logic and Bit Operations/Compare To Constant  Description=|  relop===  const=PG_ES_EngStart  OutDataTypeStr=uint8
      | 起动：只判断一个条件
      | 
      | 把输入与1比较，使用关系“==”。成立输出1，不成立输出0；输出是判断标志，不是把输入缩放成该常数。
      | 
      | 这里比较的是发动机当前模式：初始0、普通起动1、闭环2、手动3、停车4。结果供父级选择对应控制/保护路径，不能用命令编号代替模式编号。
  超转保护 : simulink/Logic and Bit Operations/Compare To Constant  Description=|  relop=>  const=62000  OutDataTypeStr=uint8
      | 超转保护：只判断一个条件
      | 
      | 把输入与62000比较，使用关系“>”。成立输出1，不成立输出0；输出是判断标志，不是把输入缩放成该常数。
      | 
      | 比较门限用于父级的分支条件，没有滤波、延时确认或锁存。例如输入恰好等于门限时，“>=、<=、==”成立，“>、<”不成立。是否需要持续确认或同时满足其他条件，由父级连线决定。
  重置指令 : simulink/Logic and Bit Operations/Compare To Constant  Description=|  relop===  const=PG_Instr_ECUReSet  OutDataTypeStr=uint8
      | 重置指令：只判断一个条件
      | 
      | 把输入与9比较，使用关系“==”。成立输出1，不成立输出0；输出是判断标志，不是把输入缩放成该常数。
      | 
      | 这里识别一种指令编码。判断成立只说明指令匹配；父级还会结合有效帧、当前模式或其他允许条件决定是否更新。实际驱动要继续经过控制与板级输出，不能把1理解为硬件执行回执。
  闭环 : simulink/Logic and Bit Operations/Compare To Constant  Description=|  relop===  const=PG_ES_Clp  OutDataTypeStr=uint8
      | 闭环：只判断一个条件
      | 
      | 把输入与2比较，使用关系“==”。成立输出1，不成立输出0；输出是判断标志，不是把输入缩放成该常数。
      | 
      | 这里比较的是发动机当前模式：初始0、普通起动1、闭环2、手动3、停车4。结果供父级选择对应控制/保护路径，不能用命令编号代替模式编号。
  S_FAM : Outport
      settings: AttributesFormatString=S_FAM（故障标志总线）
  wires:
  Bus Creator1/1 -> S_FAM/1
  S_SPM/1 -> Bus Selector1/1, Bus Selector2/1, Subsystem/1(In1)
  S_EngineState/1 -> 起动/1, 闭环/1, 手动/1, 初始状态/1, 停车状态/1, Subsystem/2(In2)
  Subsystem/2(Flag_NcFailure1) -> Bus Creator1/2  "Flag_NcFailure（转速传感器故障标志）"
  Subsystem/3(Flag_ECUReset_work) -> Bus Creator1/3  "Flag_ECUReset_work（复位恢复运行标志）"
  Subsystem/4(Flag_ECUReset_Clear) -> Bus Creator1/4  "Flag_ECUReset_Clear（清除复位恢复状态请求）"
  Subsystem/5(Flag_ECUReset_Save) -> Bus Creator1/5  "Flag_ECUReset_Save（保存复位恢复数据请求）"
  初始状态/1 -> Logical Operator1/1
  停车状态/1 -> Logical Operator1/2
  Logical Operator1/1 -> Logical Operator2/2
  Bus Selector2/1 -> 重置指令/1  "<Instr（控制指令）>"
  重置指令/1 -> Logical Operator2/3
  Logical Operator2/1 -> Data Type Conversion2/1
  Data Type Conversion2/1 -> Bus Creator1/7  "Flag_Reset_Enable（软件复位请求）"
  Bus Selector1/1 -> 超转保护/1  "<Nc_Filter（滤波后转速）>"
  超转保护/1 -> Bus Creator1/8  "OverSpeed_Protect（超转保护）"
  起动/1 -> Logical Operator3/1
  闭环/1 -> Logical Operator3/2
  手动/1 -> Logical Operator3/3
  Logical Operator3/1 -> Up_Hold/1(In)
  Up_Hold/1(Out) -> Data Type Conversion1/1, Logical Operator2/1
  Data Type Conversion1/1 -> Bus Creator1/6  "Flag_UnableCool（冷却不足标志）"
  Subsystem/1(Lock_NcFailure) -> Bus Creator1/1  "Lock_NcFailure（转速故障锁存）"

== system turbo_controller/FRAM_Read_读取恢复 ==
  note: 在发送允许时完成67字节FRAM读写传输
      |
      | 输入为Step06生成的67字节SPI帧。Enable允许时才执行SPI2传输；读帧先发送03和两字节地址，再用6
      | 4个占位字节产生时钟，返回帧中的后64字节才是记录。
      |
      | 该接口也用于整条记录写入：写帧为02、地址高、地址低和64字节数据。SPI采用模式3。返回帧经上层
      | 延迟交事务模块检查，不在本模块判断CRC或决定恢复。
      |
      | 名称含“读取恢复”，但实际帧的操作码决定读还是写；不能只凭模块名称认定其永远只读。没有使能
      | 时不会每拍重新访问FRAM。
  In1 : Inport
  Enable : EnablePort
  SPI2_FRAM_模式三传输 : stm32blockslib/SPI Controller Transfer  SPIModuleSelect=SPI2  ClockPolarity=High  ClockPhase=2 Edge  SPIModule=uint32(0)  Mode=Master  BusSpeed=uint32(1000000)  FirstBitToTransfer=Most significant bit (MSB)  ClockMode=0  BlockFunction=Transfer  EnableRegisterAddress=off  RegisterAddress=0  OutputDataType=uint8  OutputDataLength=1  OutputStatus=off  BlockingMode=on  Timeout=0.001  DataBits=8  UseCustomSSPin=Explicit GPIO calls  ActiveLowSSPin=Active low  Port_Select=GPIOB  Pin=12
      settings: LibrarySourceBlock=stm32f4xxblockslib/SPI Controller Transfer
  Out1 : Outport
  wires:
  SPI2_FRAM_模式三传输/1 -> Out1/1
  In1/1 -> SPI2_FRAM_模式三传输/1

== system turbo_controller/FRAM_写使能命令 ==
  note: 给FRAM发送一字节写使能命令
      |
      | Enable有效时，通过SPI2模式3发送输入的单字节命令，正常为06。FRAM后续的写入需要先取得写许可
      | ，因此事务层会在失效、整条记录写入、提交标志写入前安排它。
      |
      | 此模块只完成写使能传输，不包含地址和数据，也不证明下一步写入成功。返回值不等于完整记录。写
      | 后是否成功，需要后面的回读与CRC检查确认。
  In1 : Inport
  Enable : EnablePort
  SPI2_FRAM_模式三传输 : stm32blockslib/SPI Controller Transfer  SPIModuleSelect=SPI2  ClockPolarity=High  ClockPhase=2 Edge  SPIModule=uint32(0)  Mode=Master  BusSpeed=uint32(1000000)  FirstBitToTransfer=Most significant bit (MSB)  ClockMode=0  BlockFunction=Transfer  EnableRegisterAddress=off  RegisterAddress=0  OutputDataType=uint8  OutputDataLength=1  OutputStatus=off  BlockingMode=on  Timeout=0.001  DataBits=8  UseCustomSSPin=Explicit GPIO calls  ActiveLowSSPin=Active low  Port_Select=GPIOB  Pin=12
      settings: LibrarySourceBlock=stm32f4xxblockslib/SPI Controller Transfer
  Out1 : Outport
  wires:
  SPI2_FRAM_模式三传输/1 -> Out1/1
  In1/1 -> SPI2_FRAM_模式三传输/1

== system turbo_controller/FRAM_四字节提交 ==
  note: 单独改写FRAM记录最后的提交字节
      |
      | 输入固定4字节：[02，地址高字节，地址低字节，写入值]。使能成立时执行一次SPI2模式3传输。地址
      | 由事务层指定为备用记录起始地址+63。
      |
      | 先写0表示“这条记录正在更新，不可用于恢复”；完整64字节写好后，再单独写165（A5）表示“可以
      | 检查并使用”。将提交单独放最后，可避免写一半的记录被误认为完整。
      |
      | 本模块不决定写0还是165，不选择备用区，也不计算CRC；这些由Step05、Step06安排。
  In1 : Inport
  Enable : EnablePort
  SPI2_FRAM_模式三传输 : stm32blockslib/SPI Controller Transfer  SPIModuleSelect=SPI2  ClockPolarity=High  ClockPhase=2 Edge  SPIModule=uint32(0)  Mode=Master  BusSpeed=uint32(1000000)  FirstBitToTransfer=Most significant bit (MSB)  ClockMode=0  BlockFunction=Transfer  EnableRegisterAddress=off  RegisterAddress=0  OutputDataType=uint8  OutputDataLength=1  OutputStatus=off  BlockingMode=on  Timeout=0.001  DataBits=8  UseCustomSSPin=Explicit GPIO calls  ActiveLowSSPin=Active low  Port_Select=GPIOB  Pin=12
      settings: LibrarySourceBlock=stm32f4xxblockslib/SPI Controller Transfer
  Out1 : Outport
  wires:
  SPI2_FRAM_模式三传输/1 -> Out1/1
  In1/1 -> SPI2_FRAM_模式三传输/1
